simulink model "viikate_rocket"  (R2026b)
settings: Solver=ode4  StopTime=inf  FixedStep=0.001
undefined symbols (not defined in the file or in its folder): Aero, e0_0, e1_0, e2_0, e3_0, gravity, I, N, Newton, Raphson, rho, rp_burn_time_s, rp_canard_area_m2, rp_canard_cl_alpha, rp_cd0, rp_clp, rp_cmq, rp_cn_alpha, rp_cnr, rp_fin_positions_m, rp_frontal_area_m2, rp_gust_seed, rp_gust_variance, rp_ignition_time_s, rp_inertia_empty_kgm2, rp_inertia_full_kgm2, rp_length_m, rp_mass_fuel_kg, rp_mass_full_kg, rp_r_cp_m, rp_roll_ref_length_m, rp_servo_rate_limit_radps, rp_servo_tau_s, rp_thrust_n, rp_thrust_scale, rp_thrust_t_s, rp_wind_model_mps, sharedaeroassertmsg, si, Vsafe, ZYX
libraries: matrix_library x1
(part 1 of 3)
settings Model: Creator=tanel  LastModifiedBy=Minh
settings DataIOCC: ReturnWorkspaceOutputs=off
settings OptimizationCC: DefaultParameterBehavior=Inlined  DifferentSizesBufferReuse=on  EfficientTunableParamExpr=on  EnhancedBackFolding=on  OptimizationCustomize=off  OptimizeBlockOrder=speed  PassReuseOutputArgsAs=Individual arguments  RemoveInternalMemoryZeroInit=on  RemoveRootLevelIOMemoryZeroInit=on
settings DebuggingCC: ParameterTunabilityLossMsg=error
settings HardwareCC: ProdHWDeviceType=Intel->x86-64 (Linux 64)
settings ModelReferenceCC: ModelReferenceMinAlgLoopOccurrences=on
settings SFSimCC: MATLABDynamicMemAlloc=off
settings RTWCC: DataTypeReplacement=CDataTypesFixedWidth  Description=Embedded Coder  GPUComputeCapability=5.0  GenCodeOnly=on  SystemTargetFile=ert.tlc  TemplateMakefile=ert_default_tmf
settings CodeAppCC: ForceParamTrailComments=on  IgnoreCustomStorageClasses=off  InsertBlockDesc=on  OperatorAnnotations=on  SFDataObjDesc=on  SimulinkDataObjDesc=on
settings ERTTargetCC: CombineSignalStateStructs=on  MaxIdInt16=INT16_MAX  MaxIdInt32=INT32_MAX  MaxIdInt64=INT64_MAX  MaxIdInt8=INT8_MAX  MaxIdUint16=UINT16_MAX  MaxIdUint32=UINT32_MAX  MaxIdUint64=UINT64_MAX  MaxIdUint8=UINT8_MAX  MinIdInt16=INT16_MIN  MinIdInt32=INT32_MIN  MinIdInt64=INT64_MIN  MinIdInt8=INT8_MIN  SupportContinuousTime=on

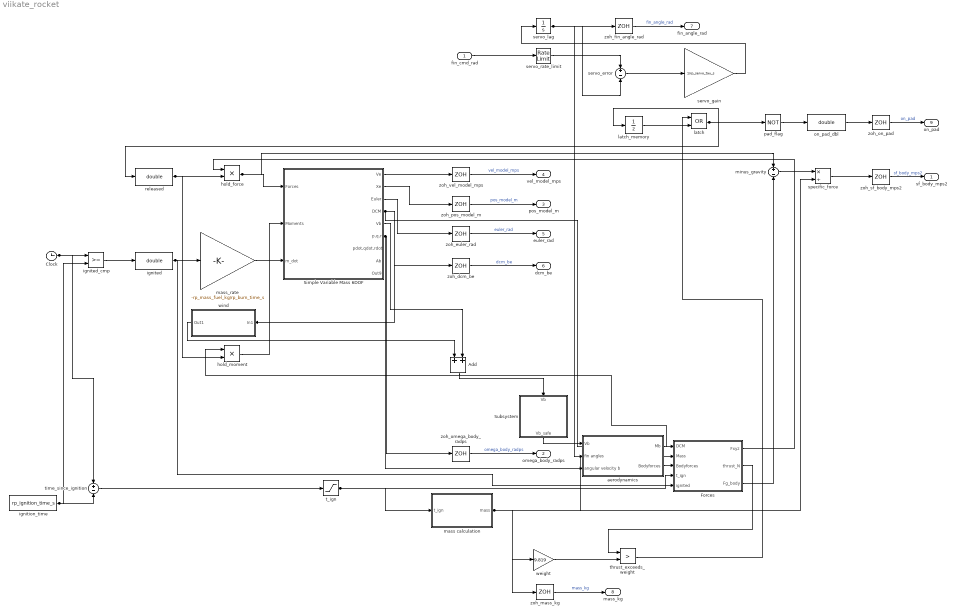
== system viikate_rocket ==
  fin_cmd_rad : Inport  OutDataTypeStr=double  PortDimensions=4  SampleTime=0.001
  Add : Sum
  Clock : Clock
  Forces : Subsystem
  Simple Variable Mass 6DOF : Subsystem  mask(6DOF EoM (Body Axis)){units=Metric (MKS), mtype=Simple Variable, rep=Quaternion, xme_0=[0 50 50], Vm_0=[0 0 0], eul_0=[0 0 0], pm_0=[0 0 0], mass_0=rp_mass_full_kg, mass_e=rp_mass_full_kg - rp_mass_fuel_kg, mass_f=rp_mass_full_kg, inertia=eye(3), inertia_e=rp_inertia_empty_kgm2, inertia_f=rp_inertia_full_kgm2, k_quat=1.0, vre_flag=off, abi_flag=off, aMode=0, xme_statename='', Vm_statename='', eul_statename='', quat_statename='', pm_statename='', mass_statename=''}
      mask prompts: units "shared_aeroblks:sharedaeroblk6dofbody:block6DOFEoMBodyAxisParamUnits"; mtype "shared_aeroblks:sharedaeroblk6dofbody:block6DOFEoMBodyAxisParamMasstype"; rep "shared_aeroblks:sharedaeroblk6dofbody:block6DOFEoMBodyAxisParamRepresentation"; xme_0 "shared_aeroblks:sharedaeroblk6dofbody:block6DOFEoMBodyAxisParamInitialpositionininertialaxesXeYeZe"; Vm_0 "shared_aeroblks:sharedaeroblk6dofbody:block6DOFEoMBodyAxisParamInitialvelocityinbodyaxesUvw"; eul_0 "shared_aeroblks:sharedaeroblk6dofbody:block6DOFEoMBodyAxisParamInitialEulerorientationrollpitchyaw"; pm_0 "shared_aeroblks:sharedaeroblk6dofbody:block6DOFEoMBodyAxisParamInitialbodyrotationratespqr"; mass_0 "shared_aeroblks:sharedaeroblk6dofbody:block6DOFEoMBodyAxisParamInitialmass"; mass_e "shared_aeroblks:sharedaeroblk6dofbody:block6DOFEoMBodyAxisParamEmptymass"; mass_f "shared_aeroblks:sharedaeroblk6dofbody:block6DOFEoMBodyAxisParamFullmass"; inertia "shared_aeroblks:sharedaeroblk6dofbody:block6DOFEoMBodyAxisParamInertia"; inertia_e "shared_aeroblks:sharedaeroblk6dofbody:block6DOFEoMBodyAxisParamEmptyinertiamatrix"; inertia_f "shared_aeroblks:sharedaeroblk6dofbody:block6DOFEoMBodyAxisParamFullinertiamatrix"; k_quat "shared_aeroblks:sharedaeroblk6dofbody:block6DOFEoMBodyAxisParamGainforquaternionnormalization"; vre_flag "shared_aeroblks:sharedaeroblk6dofbody:block6DOFEoMBodyAxisParamIncludemassflowrelativevelocity"; abi_flag "shared_aeroblks:sharedaeroblk6dofbody:inertialAccelFlag"; xme_statename "shared_aeroblks:sharedaeroblk6dofbody:block6DOFEoMStateNamePosition"; Vm_statename "shared_aeroblks:sharedaeroblk6dofbody:block6DOFEoMStateNameVelocity"; eul_statename "shared_aeroblks:sharedaeroblk6dofbody:block6DOFEoMStateNameEulerAngles"; quat_statename "shared_aeroblks:sharedaeroblk6dofbody:block6DOFEoMStateNameQuaternions"; pm_statename "shared_aeroblks:sharedaeroblk6dofbody:block6DOFEoMStateNameRotationRates"; mass_statename "shared_aeroblks:sharedaeroblk6dofbody:block6DOFEoMStateNameMass"
      mask help: shared_aeroblks:sharedaeroblk6dofbody:block6DOFEoMBodyAxisDesc
      mask init:
      | if aerosharedtest(gcb)
      |     ports=aerosharedicon('shared6dofbody','icon');
      | else
      |     ports=sharedautoicon('shared6dofbody','icon');
      | end
      mask Help: eval('aerosharedhelp(''simple_variable_mass_6dof_quaternion'')');
      mask TypeOptions units: shared_aeroblks:sharedaeroblk6dofbody:block6DOFEoMBodyAxisParamComboMetricMKS | shared_aeroblks:sharedaeroblk6dofbody:block6DOFEoMBodyAxisParamComboEnglishVelocityinfts | shared_aeroblks:sharedaeroblk6dofbody:block6DOFEoMBodyAxisParamComboEnglishVelocityinkts
      mask TypeOptions mtype: shared_aeroblks:sharedaeroblk6dofbody:block6DOFEoMBodyAxisParamComboFixed | shared_aeroblks:sharedaeroblk6dofbody:block6DOFEoMBodyAxisParamComboSimpleVariable | shared_aeroblks:sharedaeroblk6dofbody:block6DOFEoMBodyAxisParamComboCustomVariable
      mask Callback mtype:
      | if aerosharedtest(gcb) && builtin('license','test','aerospace_blockset')
      |     aerosharedicon('shared6dofbody');
      | else
      |     sharedautoicon('shared6dofbody');
      | end
      mask TypeOptions rep: shared_aeroblks:sharedaeroblk6dofbody:block6DOFEoMBodyAxisParamComboEulerAngles | shared_aeroblks:sharedaeroblk6dofbody:block6DOFEoMBodyAxisParamComboQuaternion
      mask Callback rep:
      | if aerosharedtest(gcb) && builtin('license','test','aerospace_blockset')
      |     aerosharedicon('shared6dofbody');
      | else
      |     sharedautoicon('shared6dofbody');
      | end
      mask DialogControl Container4 Prompt: shared_aeroblks:sharedaeroblk6dofbody:block6DOFEoMParamTab
      mask DialogControl units Prompt: Units:
      mask DialogControl mtype Prompt: Mass type:
      mask DialogControl rep Prompt: Representation:
      mask DialogControl xme_0 Prompt: Initial position in inertial axes [Xe,Ye,Ze]:
      mask DialogControl Vm_0 Prompt: Initial velocity in body axes [U,v,w]:
      mask DialogControl eul_0 Prompt: Initial Euler orientation [roll, pitch, yaw]:
      mask DialogControl pm_0 Prompt: Initial body rotation rates [p,q,r]:
      mask DialogControl mass_0 Prompt: Initial mass:
      mask DialogControl mass_e Prompt: Empty mass:
      mask DialogControl mass_f Prompt: Full mass:
      mask DialogControl inertia Prompt: Inertia:
      mask DialogControl inertia_e Prompt: Empty inertia matrix:
      mask DialogControl inertia_f Prompt: Full inertia matrix:
      mask DialogControl k_quat Prompt: Gain for quaternion normalization:
      mask DialogControl vre_flag Prompt: Include mass flow relative velocity
      mask DialogControl abi_flag Prompt: Include inertial acceleration
      mask DialogControl Container6 Prompt: shared_aeroblks:sharedaeroblk6dofbody:block6DOFEoMStateAttributesTab
      mask DialogControl Container7 Prompt: shared_aeroblks:sharedaeroblk6dofbody:block6DOFEoMStateNamesGroup
      mask DialogControl xme_statename Prompt: Position: e.g., {'Xe', 'Ye', 'Ze'}
      mask DialogControl Vm_statename Prompt: Velocity: e.g., {'U', 'v', 'w'}
      mask DialogControl eul_statename Prompt: Euler rotation angles: e.g., {'phi', 'theta', 'psi'}
      mask DialogControl quat_statename Prompt: Quaternion vector: e.g., {'qr', 'qi', 'qj', 'qk'}
      mask DialogControl pm_statename Prompt: Body rotation rates: e.g., {'p', 'q', 'r'}
      mask DialogControl mass_statename Prompt: Mass: e.g., 'mass'
      mask Display:
      | port_label(ports(1).type,ports(1).port,ports(1).txt,'texmode','on');
      | port_label(ports(2).type,ports(2).port,ports(2).txt,'texmode','on');
      | port_label(ports(3).type,ports(3).port,ports(3).txt,'texmode','on');
      | port_label(ports(4).type,ports(4).port,ports(4).txt,'texmode','on');
      | port_label(ports(5).type,ports(5).port,ports(5).txt,'texmode','on');
      | port_label(ports(6).type,ports(6).port,ports(6).txt,'texmode','on');
      | port_label(ports(7).type,ports(7).port,ports(7).txt,'texmode','on');
      | port_label(ports(8).type,ports(8).port,ports(8).txt,'texmode','on');
      | port_label(ports(9).type,ports(9).port,ports(9).txt,'texmode','on');
      | port_label(ports(10).type,ports(10).port,ports(10).txt,'texmode','on');
      | port_label(ports(11).type,ports(11).port,ports(11).txt,'texmode','on');
      | port_label(ports(12).type,ports(12).port,ports(12).txt,'texmode','on');
      | port_label(ports(13).type,ports(13).port,ports(13).txt,'texmode','on');
      | port_label(ports(14).type,ports(14).port,ports(14).txt,'texmode','on');
      | port_label(ports(15).type,ports(15).port,ports(15).txt,'texmode','on');
      | port_label(ports(16).type,ports(16).port,ports(16).txt,'texmode','on');
      | port_label(ports(17).type,ports(17).port,ports(17).txt,'texmode','on');
  Subsystem : Subsystem
  aerodynamics : Subsystem
  hold_force : Product
  hold_moment : Product
  ignited : DataTypeConversion  OutDataTypeStr=double  SaturateOnIntegerOverflow=off  RndMeth=Floor
  ignited_cmp : RelationalOperator  OutDataTypeStr=boolean  ZeroCross=off  RndMeth=Simplest  InputSameDT=off
  ignition_time : Constant  Value=rp_ignition_time_s
  latch : Logic  Operator=OR  AllPortsSameDT=off  OutDataTypeStr=boolean
  latch_memory : UnitDelay  InitialCondition=false  SampleTime=0.001
  mass calculation : Subsystem
  mass_rate : Gain  Gain=-rp_mass_fuel_kg/rp_burn_time_s
  minus_gravity : Sum  Inputs=+-
  on_pad_dbl : DataTypeConversion  OutDataTypeStr=double  SaturateOnIntegerOverflow=off  RndMeth=Floor
  pad_flag : Logic  Operator=NOT  AllPortsSameDT=off  OutDataTypeStr=boolean
  released : DataTypeConversion  OutDataTypeStr=double  SaturateOnIntegerOverflow=off  RndMeth=Floor
  servo_error : Sum  Inputs=+-
  servo_gain : Gain  Gain=1/rp_servo_tau_s
  servo_lag : Integrator
  servo_rate_limit : RateLimiter  RisingSlewLimit=rp_servo_rate_limit_radps  FallingSlewLimit=-rp_servo_rate_limit_radps  SampleTimeMode=inherited
  specific_force : Product  Inputs=*/
  t_ign : Saturate  UpperLimit=inf  LowerLimit=0  ZeroCross=off
  thrust_exceeds_weight : RelationalOperator  Operator=>  OutDataTypeStr=boolean  SampleTime=0.001  RndMeth=Simplest  InputSameDT=off
  time_since_ignition : Sum  Inputs=+-
  weight : Gain  Gain=9.819
  wind : Subsystem
  zoh_dcm_be : ZeroOrderHold  SampleTime=0.001
  zoh_euler_rad : ZeroOrderHold  SampleTime=0.001
  zoh_fin_angle_rad : ZeroOrderHold  SampleTime=0.001
  zoh_mass_kg : ZeroOrderHold  SampleTime=0.001
  zoh_omega_body_radps : ZeroOrderHold  SampleTime=0.001
  zoh_on_pad : ZeroOrderHold  SampleTime=0.001
  zoh_pos_model_m : ZeroOrderHold  SampleTime=0.001
  zoh_sf_body_mps2 : ZeroOrderHold  SampleTime=0.001
  zoh_vel_model_mps : ZeroOrderHold  SampleTime=0.001
  sf_body_mps2 : Outport
  omega_body_radps : Outport  Port=2
  pos_model_m : Outport  Port=3
  vel_model_mps : Outport  Port=4
  euler_rad : Outport  Port=5
  dcm_be : Outport  Port=6
  fin_angle_rad : Outport  Port=7
  mass_kg : Outport  Port=8
  on_pad : Outport  Port=9
  wires:
  minus_gravity/1 -> specific_force/1
  pad_flag/1 -> on_pad_dbl/1
  Forces/1(Fxyz) -> hold_force/1
  latch/1 -> pad_flag/1, released/1, latch_memory/1
  thrust_exceeds_weight/1 -> latch/1
  aerodynamics/2(Bodyforces) -> Forces/3(Bodyforces)
  aerodynamics/1(Mb) -> hold_moment/1
  zoh_fin_angle_rad/1 -> fin_angle_rad/1  "fin_angle_rad"
  zoh_mass_kg/1 -> mass_kg/1  "mass_kg"
  Simple Variable Mass 6DOF/1(Ve) -> zoh_vel_model_mps/1
  zoh_on_pad/1 -> on_pad/1  "on_pad"
  Simple Variable Mass 6DOF/2(Xe) -> zoh_pos_model_m/1
  ignition_time/1 -> ignited_cmp/2, time_since_ignition/2
  Simple Variable Mass 6DOF/6(p,q,r) -> zoh_omega_body_radps/1, aerodynamics/3(angular velocity b)
  mass_rate/1 -> Simple Variable Mass 6DOF/3(m_dot)
  hold_force/1 -> Simple Variable Mass 6DOF/1(Forces), minus_gravity/1
  ignited/1 -> mass_rate/1, Forces/5(ignited)
  servo_gain/1 -> servo_lag/1
  time_since_ignition/1 -> t_ign/1
  released/1 -> hold_moment/2, hold_force/2
  Simple Variable Mass 6DOF/3(Euler) -> zoh_euler_rad/1
  Add/1 -> Subsystem/1(Vb)
  on_pad_dbl/1 -> zoh_on_pad/1
  Forces/3(Fg_body) -> minus_gravity/2
  zoh_dcm_be/1 -> dcm_be/1  "dcm_be"
  Clock/1 -> ignited_cmp/1, time_since_ignition/1
  hold_moment/1 -> Simple Variable Mass 6DOF/2(Moments)
  servo_rate_limit/1 -> servo_error/1
  latch_memory/1 -> latch/2
  wind/1(Out1) -> Add/1
  Simple Variable Mass 6DOF/4(DCM) -> zoh_dcm_be/1, Forces/1(DCM), wind/1(In1)
  Simple Variable Mass 6DOF/5(Vb) -> Add/2
  zoh_sf_body_mps2/1 -> sf_body_mps2/1  "sf_body_mps2"
  t_ign/1 -> mass calculation/1(t_ign), Forces/4(t_ign)
  servo_error/1 -> servo_gain/1
  fin_cmd_rad/1 -> servo_rate_limit/1
  specific_force/1 -> zoh_sf_body_mps2/1
  Subsystem/1(Vb_safe) -> aerodynamics/1(Vb)
  zoh_vel_model_mps/1 -> vel_model_mps/1  "vel_model_mps"
  zoh_pos_model_m/1 -> pos_model_m/1  "pos_model_m"
  zoh_euler_rad/1 -> euler_rad/1  "euler_rad"
  zoh_omega_body_radps/1 -> omega_body_radps/1  "omega_body_radps"
  Forces/2(thrust_N) -> thrust_exceeds_weight/1
  mass calculation/1(mass) -> zoh_mass_kg/1, weight/1, Forces/2(Mass), specific_force/2
  servo_lag/1 -> zoh_fin_angle_rad/1, aerodynamics/2(fin angles), servo_error/2
  ignited_cmp/1 -> ignited/1
  weight/1 -> thrust_exceeds_weight/2

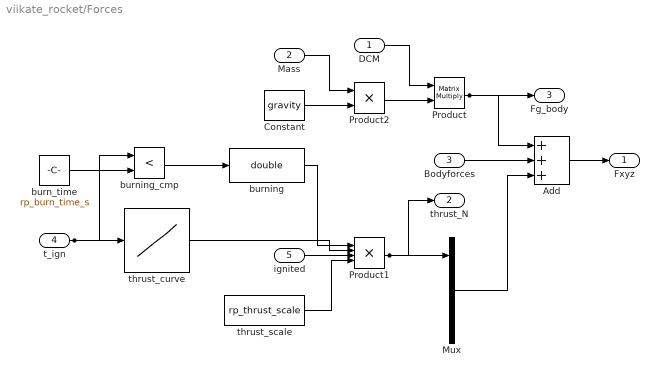
== system viikate_rocket/Forces ==
  DCM : Inport
  Mass : Inport  Port=2
  Bodyforces : Inport  Port=3
  t_ign : Inport  Port=4
  ignited : Inport  Port=5
  Add : Sum  Inputs=+|+|+
  Constant : Constant  Value=gravity  VectorParams1D=off
  Mux : Mux  Inputs=3
  Product : Product  Multiplication=Matrix(*)
  Product1 : Product  Inputs=4
  Product2 : Product
  burn_time : Constant  Value=rp_burn_time_s
  burning : DataTypeConversion  OutDataTypeStr=double  SaturateOnIntegerOverflow=off  RndMeth=Floor
  burning_cmp : RelationalOperator  Operator=<  OutDataTypeStr=boolean  ZeroCross=off  RndMeth=Simplest  InputSameDT=off
  thrust_curve : Lookup_n-D  NumberOfTableDimensions=1  BreakpointsForDimension1=rp_thrust_t_s  Table=rp_thrust_n  ExtrapMethod=Clip  InternalRulePriority=Speed  RndMeth=Simplest
  thrust_scale : Constant  Value=rp_thrust_scale
  Fxyz : Outport
  thrust_N : Outport  Port=2
  Fg_body : Outport  Port=3
  wires:
  Add/1 -> Fxyz/1
  Mux/1 -> Add/3
  burn_time/1 -> burning_cmp/2
  burning/1 -> Product1/1
  Bodyforces/1 -> Add/2
  t_ign/1 -> burning_cmp/1, thrust_curve/1
  Product1/1 -> thrust_N/1, Mux/1
  Product/1 -> Fg_body/1, Add/1
  burning_cmp/1 -> burning/1
  Mass/1 -> Product2/1
  Product2/1 -> Product/2
  Constant/1 -> Product2/2
  thrust_curve/1 -> Product1/2
  ignited/1 -> Product1/3
  thrust_scale/1 -> Product1/4
  DCM/1 -> Product/1

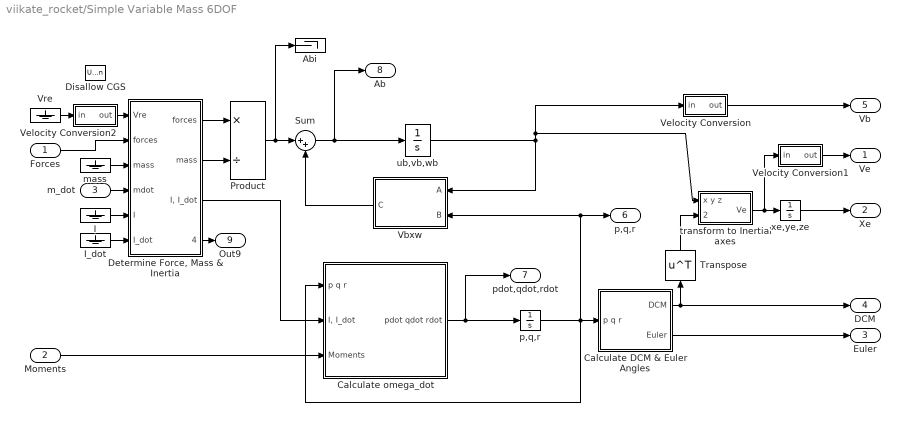
== system viikate_rocket/Simple Variable Mass 6DOF ==
  Forces : Inport  OutDataTypeStr=double  Unit=N  PortDimensions=3
  Moments : Inport  Port=2  OutDataTypeStr=double  Unit=N*m  PortDimensions=3
  m_dot : Inport  Port=3  Unit=kg/s
  Abi : Terminator
  Calculate DCM & Euler Angles : Subsystem  mask(DCM & Euler Angles (Quaternion)){aMode=aMode}
      mask init:
      | if aerosharedtest(gcb)
      |     aerosharedicon('shared');
      | else
      |     sharedautoicon('shared');
      | end
  Calculate omega_dot : Subsystem  mask{aMode=aMode}
      mask init:
      | if aerosharedtest(gcb)
      |     aerosharedicon('shared');
      | else
      |     sharedautoicon('shared');
      | end
  "Determine Force, Mass & Inertia" : Subsystem  mask(Mass & Inertia (simple)){aMode=aMode}
      mask init:
      | if aerosharedtest(gcb)
      |     aerosharedicon('shared');
      | else
      |     sharedautoicon('shared');
      | end
  Disallow CGS : UnitConfiguration  UnitSystemsStr=English,SI,SI (extended)  AllowAllUnitSystems=off
  I : Ground
  I_dot : Ground
  Product : Product  Inputs=*/  SaturateOnIntegerOverflow=on  OutDataTypeStr=Inherit: Same as first input
  Sum : Sum  Inputs=|++  SaturateOnIntegerOverflow=on
  Transpose : Math  Operator=transpose  SignedPower=on
  Vbxw : Subsystem  mask(CrossProduct){aMode=aMode}
      mask help: shared_aeroblks:sharedaeroblkutil:blockCrossProductDesc
      mask init:
      | if aerosharedtest(gcb)
      |     aerosharedicon('shared');
      | else
      |     sharedautoicon('shared');
      | end
      mask Help: eval('if license(''test'',''Aerospace_Blockset'')aerosharedhelp(''threebythree_cross_product'');elseif license(''test'',''Powertrain_Blockset'')sharedautohelp(''threebythree_cross_product'');end')
      mask Display:
      | text(.5,.5,'Cross\nProduct\nC = AxB', ...
      | 	'HorizontalAlignment','Center',...
      | 	'VerticalAlignment','middle')
  Velocity Conversion : Subsystem
  Velocity Conversion1 : Subsystem
  Velocity Conversion2 : Subsystem
  Vre : Ground
  mass : Ground
  "p,q,r " : Integrator  InitialCondition=pm_0  ContinuousStateAttributes=pm_statename
  "transform to Inertial axes " : Subsystem  mask(Vector Transformation){}
      mask Display: disp('L_EB')
  ub,vb,wb : Integrator  InitialCondition=Vm_0  ContinuousStateAttributes=Vm_statename
  xe,ye,ze : Integrator  InitialCondition=xme_0  ContinuousStateAttributes=xme_statename
  Ve : Outport  OutDataTypeStr=double  Unit=m/s  VectorParamsAs1DForOutWhenUnconnected=off
  Xe : Outport  Port=2  OutDataTypeStr=double  Unit=m  VectorParamsAs1DForOutWhenUnconnected=off
  Euler : Outport  Port=3  OutDataTypeStr=double  Unit=rad  VectorParamsAs1DForOutWhenUnconnected=off
  DCM : Outport  Port=4  OutDataTypeStr=double  Unit=1  VectorParamsAs1DForOutWhenUnconnected=off
  Vb : Outport  Port=5  OutDataTypeStr=double  Unit=m/s  VectorParamsAs1DForOutWhenUnconnected=off
  p,q,r : Outport  Port=6  OutDataTypeStr=double  Unit=rad/s  VectorParamsAs1DForOutWhenUnconnected=off
  pdot,qdot,rdot : Outport  Port=7  OutDataTypeStr=double  Unit=rad/s^2  VectorParamsAs1DForOutWhenUnconnected=off
  Ab : Outport  Port=8  OutDataTypeStr=double  Unit=m/s^2  VectorParamsAs1DForOutWhenUnconnected=off
  Out9 : Outport  Port=9  Unit=1
  wires:
  Velocity Conversion1/1(out) -> Ve/1
  Sum/1 -> Ab/1, ub,vb,wb/1
  ub,vb,wb/1 -> Vbxw/1(A), Velocity Conversion/1(in), "transform to Inertial axes "/1(x y z)
  Velocity Conversion/1(out) -> Vb/1
  Velocity Conversion2/1(out) -> "Determine Force, Mass & Inertia"/1(Vre)
  Vre/1 -> Velocity Conversion2/1(in)
  "Determine Force, Mass & Inertia"/1("forces ") -> Product/1
  I_dot/1 -> "Determine Force, Mass & Inertia"/6(I_dot)
  I/1 -> "Determine Force, Mass & Inertia"/5(I)
  Calculate omega_dot/1(pdot qdot rdot) -> "p,q,r "/1, pdot,qdot,rdot/1
  "Determine Force, Mass & Inertia"/4(tank limit) -> Out9/1
  m_dot/1 -> "Determine Force, Mass & Inertia"/4(mdot)
  "Determine Force, Mass & Inertia"/2(mass) -> Product/2
  mass/1 -> "Determine Force, Mass & Inertia"/3("mass ")
  Transpose/1 -> "transform to Inertial axes "/2(transform coefficients)
  Calculate DCM & Euler Angles/1(DCM) -> Transpose/1, DCM/1
  Product/1 -> Sum/1, Abi/1
  Forces/1 -> "Determine Force, Mass & Inertia"/2(forces)
  Moments/1 -> Calculate omega_dot/3(Moments)
  "p,q,r "/1 -> Calculate DCM & Euler Angles/1(p q r), Calculate omega_dot/1(p q r), p,q,r/1, Vbxw/2(B)
  "transform to Inertial axes "/1(Ve) -> xe,ye,ze/1, Velocity Conversion1/1(in)
  xe,ye,ze/1 -> Xe/1
  Vbxw/1(C) -> Sum/2
  Calculate DCM & Euler Angles/2(Euler) -> Euler/1
  "Determine Force, Mass & Inertia"/3("I, I_dot") -> Calculate omega_dot/2("I, I_dot")

== system viikate_rocket/Subsystem ==
  Vb : Inport
  Abs : Abs  SaturateOnIntegerOverflow=off
  Constant3 : Constant  Value=Vsafe
  Demux : Demux  Outputs=3
  Mux : Mux  Inputs=3
  Switch2 : Switch  Threshold=Vsafe  SaturateOnIntegerOverflow=off  InputSameDT=off
  Vb_safe : Outport
  wires:
  Vb/1 -> Demux/1
  Abs/1 -> Switch2/2
  Demux/2 -> Mux/2
  Demux/3 -> Mux/3
  Switch2/1 -> Mux/1
  Mux/1 -> Vb_safe/1
  Demux/1 -> Switch2/1, Abs/1
  Constant3/1 -> Switch2/3

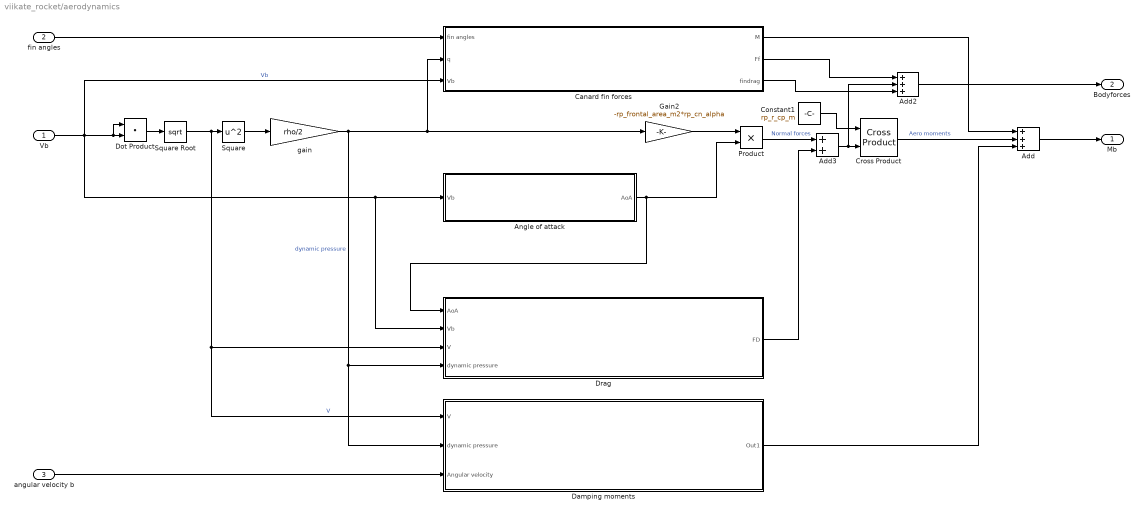
== system viikate_rocket/aerodynamics ==
  Vb : Inport
  fin angles : Inport  Port=2
  angular velocity b : Inport  Port=3
  Add : Sum  Inputs=+++
  Add2 : Sum  Inputs=+++
  Add3 : Sum
  Angle of attack : Subsystem
  Canard fin forces : Subsystem
  Constant1 : Constant  Value=rp_r_cp_m
  Cross Product : matrix_library/Cross Product
  Damping moments : Subsystem
  Dot Product : DotProduct  OutDataTypeStr=Inherit: Inherit via internal rule
  Drag : Subsystem
  Gain2 : Gain  Gain=-rp_frontal_area_m2*rp_cn_alpha
  Product : Product
  Square : Math  Operator=square
  Square Root : Sqrt
  gain : Gain  Gain=rho/2
  Mb : Outport
  Bodyforces : Outport  Port=2
  wires:
  Gain2/1 -> Product/1
  Constant1/1 -> Cross Product/1
  Product/1 -> Add3/1  "Normal forces"
  Cross Product/1 -> Add/2  "Aero moments"
  Add/1 -> Mb/1
  Add2/1 -> Bodyforces/1
  Canard fin forces/2(Ff) -> Add2/1
  Add3/1 -> Add2/2, Cross Product/2
  Vb/1 -> Canard fin forces/3(Vb), Dot Product/1, Dot Product/2, Angle of attack/1(Vb), Drag/2(Vb)  "Vb"
  Square/1 -> gain/1
  Square Root/1 -> Damping moments/1(V), Drag/3(V), Square/1  "V"
  Dot Product/1 -> Square Root/1
  gain/1 -> Damping moments/2(dynamic pressure), Drag/4(dynamic pressure), Canard fin forces/2(q), Gain2/1  "dynamic pressure"
  fin angles/1 -> Canard fin forces/1(fin angles)
  Canard fin forces/1(M) -> Add/1
  Drag/1(FD) -> Add3/2
  Angle of attack/1(AoA) -> Product/2, Drag/1(AoA)
  angular velocity b/1 -> Damping moments/3(Angular velocity)
  Damping moments/1(Out1) -> Add/3
  Canard fin forces/3(findrag) -> Add2/3

== system viikate_rocket/mass calculation ==
  t_ign : Inport
  Add : Sum
  Constant1 : Constant  Value=rp_mass_full_kg
  Constant2 : Constant  Value=-rp_mass_fuel_kg/rp_burn_time_s
  Product : Product
  Saturation : Saturate  UpperLimit=rp_mass_full_kg  LowerLimit=rp_mass_full_kg - rp_mass_fuel_kg
  mass : Outport
  wires:
  Add/1 -> Saturation/1
  Product/1 -> Add/2
  Saturation/1 -> mass/1
  t_ign/1 -> Product/2
  Constant1/1 -> Add/1
  Constant2/1 -> Product/1

== system viikate_rocket/wind ==
  In1 : Inport
  Constant3 : Constant  Value=0
  Gain : Gain  Gain=-1
  Integrator : Integrator  InitialCondition=rp_wind_model_mps
  Matrix Multiply : Product  Multiplication=Matrix(*)
  Mux : Mux  Inputs=3
  Random Number1 : RandomNumber  Variance=rp_gust_variance  Seed=rp_gust_seed(1)  SampleTime=0.01
  Random Number2 : RandomNumber  Variance=rp_gust_variance  Seed=rp_gust_seed(2)  SampleTime=0.01
  Out1 : Outport
  wires:
  Mux/1 -> Integrator/1
  Constant3/1 -> Mux/1
  Gain/1 -> Matrix Multiply/2
  Random Number1/1 -> Mux/2
  Random Number2/1 -> Mux/3
  Integrator/1 -> Gain/1
  Matrix Multiply/1 -> Out1/1
  In1/1 -> Matrix Multiply/1

== system viikate_rocket/Simple Variable Mass 6DOF/Calculate DCM & Euler Angles ==
  p q r : Inport  OutDataTypeStr=double
  Initial Euler Angles : Constant  Value=eul_0
  Quaternions to Direction Cosine Matrix : Subsystem  mask(Quaternion2DCM){aMode=aMode}
      mask help: shared_aeroblks:sharedaeroblktransform:blockQuaternion2DCMDesc
      mask init:
      | if aerosharedtest(gcb)
      |     ports=aerosharedicon('shared');
      | else
      |     ports=sharedautoicon('shared');
      | end
      mask Help: eval('if license(''test'',''Aerospace_Blockset'')aerosharedhelp(''quaternions_to_direction_cosine_matrix'');elseif license(''test'',''Powertrain_Blockset'')sharedautohelp(''quaternions_to_direction_cosine_matrix'');end')
      mask Display:
      | port_label('input',1,'q','texmode','on')
      | port_label('output',1,'DCM_{be}','texmode','on')
  Quaternions to Rotation Angles : Subsystem  mask(Quat2Ang){rotationOrder=ZYX, aMode=aMode}
      mask prompts: rotationOrder "shared_aeroblks:sharedaeroblktransform:blockDCM2AngParamRotationOrder"
      mask help: shared_aeroblks:sharedaeroblktransform:blockQuat2AngDesc
      settings: AttributesFormatString=Rotation Order: %<rotationOrder>
      mask Help: eval('if license(''test'',''Aerospace_Blockset'')aerosharedhelp(''quaternions_to_rotation_angles'');elseif license(''test'',''Powertrain_Blockset'')sharedautohelp(''quaternions_to_rotation_angles'');end')
      mask TypeOptions rotationOrder: DCM2Ang/rotationOrder
      mask DialogControl rotationOrder Prompt: Rotation order:
      mask Display:
      | port_label('input',1,'q','texmode','on')
      | port_label('output',1,'[R_1,R_2,R_3]','texmode','on')
  Rotation Angles to Quaternions : Subsystem  mask(Ang2Quat){rotationOrder=ZYX, aMode=aMode}
      mask prompts: rotationOrder "shared_aeroblks:sharedaeroblktransform:blockAng2QuatParamRotationOrder"
      mask help: shared_aeroblks:sharedaeroblktransform:blockAng2QuatDesc
      mask init:
      | if aerosharedtest(gcb)
      |     ports=aerosharedicon('sharedang2quat');
      | else
      |     ports=sharedautoicon('sharedang2quat');
      | end
      settings: AttributesFormatString=Rotation Order: %<rotationOrder>
      mask Help: eval('if license(''test'',''Aerospace_Blockset'')aerosharedhelp(''rotation_angles_to_quaternions'');elseif license(''test'',''Powertrain_Blockset'')sharedautohelp(''rotation_angles_to_quaternions'');end')
      mask TypeOptions rotationOrder: shared_aeroblks:sharedaeroblktransform:blockParamComboZYX | shared_aeroblks:sharedaeroblktransform:blockParamComboZYZ | shared_aeroblks:sharedaeroblktransform:blockParamComboZXY | shared_aeroblks:sharedaeroblktransform:blockParamComboZXZ | shared_aeroblks:sharedaeroblktransform:blockParamComboYXZ | shared_aeroblks:sharedaeroblktransform:blockParamComboYXY | shared_aeroblks:sharedaeroblktransform:blockParamComboYZX | shared_aeroblks:sharedaeroblktransform:blockParamComboYZY | shared_aeroblks:sharedaeroblktransform:blockParamComboXYZ | shared_aeroblks:sharedaeroblktransform:blockParamComboXYX | shared_aeroblks:sharedaeroblktransform:blockParamComboXZY | shared_aeroblks:sharedaeroblktransform:blockParamComboXZX
      mask DialogControl rotationOrder Prompt: Rotation order:
      mask Display:
      | port_label('input',1,'[R_1,R_2,R_3]','texmode','on')
      | port_label('output',1,'q','texmode','on')
  Selector : Selector  InputPortWidth=3  IndexOptions=Index vector (dialog)  Indices=[3 2 1]  OutputSizes=1  RuntimeRangeChecks=off
  Selector1 : Selector  InputPortWidth=3  IndexOptions=Index vector (dialog)  Indices=[3 2 1]  OutputSizes=1  RuntimeRangeChecks=off
  q0 q1 q2 q3 : Integrator  InitialConditionSource=external  InitialCondition=[e0_0 e1_0 e2_0 e3_0]  ContinuousStateAttributes=quat_statename
  qdot : Subsystem
  DCM : Outport  OutDataTypeStr=double  VectorParamsAs1DForOutWhenUnconnected=off
  Euler : Outport  Port=2  OutDataTypeStr=double  VectorParamsAs1DForOutWhenUnconnected=off
  wires:
  Selector1/1 -> Rotation Angles to Quaternions/1("R1, R2, R3")
  Selector/1 -> Euler/1
  Quaternions to Rotation Angles/1(R1,R2,R3) -> Selector/1
  Quaternions to Direction Cosine Matrix/1(DCM) -> DCM/1
  p q r/1 -> qdot/1(p q r)
  Initial Euler Angles/1 -> Selector1/1
  Rotation Angles to Quaternions/1(Quat) -> q0 q1 q2 q3/2
  q0 q1 q2 q3/1 -> qdot/2(q0 q1 q2 q3), Quaternions to Rotation Angles/1(q), Quaternions to Direction Cosine Matrix/1(Quat)
  qdot/1(qdot) -> q0 q1 q2 q3/1

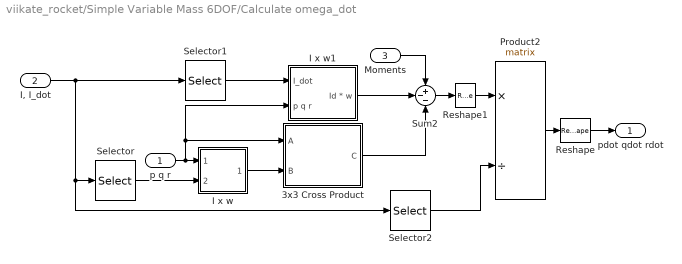
== system viikate_rocket/Simple Variable Mass 6DOF/Calculate omega_dot ==
  p q r : Inport  OutDataTypeStr=double
  "I, I_dot" : Inport  Port=2  OutDataTypeStr=double
  Moments : Inport  Port=3  OutDataTypeStr=double
  3x3 Cross Product : Subsystem  mask(CrossProduct){aMode=aMode}
      mask help: shared_aeroblks:sharedaeroblkutil:blockCrossProductDesc
      mask init:
      | if aerosharedtest(gcb)
      |     aerosharedicon('shared');
      | else
      |     sharedautoicon('shared');
      | end
      mask Help: eval('if license(''test'',''Aerospace_Blockset'')aerosharedhelp(''threebythree_cross_product'');elseif license(''test'',''Powertrain_Blockset'')sharedautohelp(''threebythree_cross_product'');end')
      mask Display:
      | text(.5,.5,'Cross\nProduct\nC = AxB', ...
      | 	'HorizontalAlignment','Center',...
      | 	'VerticalAlignment','middle')
  I x w : Subsystem
  I x w1 : Subsystem
  Product2 : Product  Inputs=*/  Multiplication=Matrix(*)  SaturateOnIntegerOverflow=on  OutDataTypeStr=Inherit: Same as first input
  Reshape : Reshape
  Reshape1 : Reshape  OutputDimensionality=Row vector (2-D)
  Selector : Selector  NumberOfDimensions=2  InputPortWidth=2  IndexOptions=Index vector (dialog),Select all  Indices=1:3,-1  OutputSizes=1  RuntimeRangeChecks=off
  Selector1 : Selector  NumberOfDimensions=2  InputPortWidth=2  IndexOptions=Index vector (dialog),Select all  Indices=4:6,-1  OutputSizes=1  RuntimeRangeChecks=off
  Selector2 : Selector  NumberOfDimensions=2  InputPortWidth=2  IndexOptions=Index vector (dialog),Select all  Indices=1:3,-1  OutputSizes=1  RuntimeRangeChecks=off
  Sum2 : Sum  Inputs=+--  SaturateOnIntegerOverflow=on
  pdot qdot rdot : Outport  OutDataTypeStr=double  VectorParamsAs1DForOutWhenUnconnected=off
  wires:
  Reshape1/1 -> Product2/1
  I x w/1(I * w) -> 3x3 Cross Product/2(B)
  3x3 Cross Product/1(C) -> Sum2/3
  Selector1/1 -> I x w1/1(I_dot)
  I x w1/1(Id * w) -> Sum2/2
  Moments/1 -> Sum2/1
  Sum2/1 -> Reshape1/1
  Product2/1 -> Reshape/1
  p q r/1 -> I x w1/2(p q r), 3x3 Cross Product/1(A), I x w/1(p q r)
  "I, I_dot"/1 -> Selector1/1, Selector2/1, Selector/1
  Selector2/1 -> Product2/2
  Selector/1 -> I x w/2(Inertia)
  Reshape/1 -> pdot qdot rdot/1

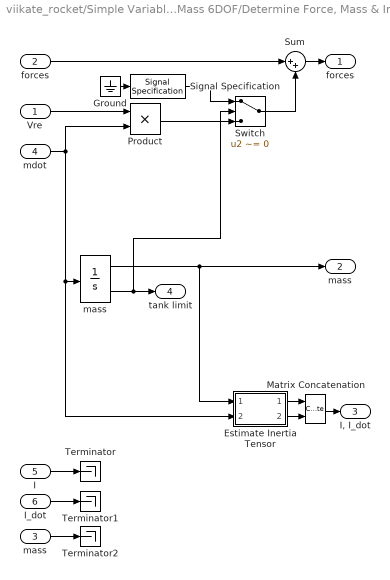
== system viikate_rocket/Simple Variable Mass 6DOF/Determine Force, Mass & Inertia ==
  Vre : Inport  OutDataTypeStr=double
  forces : Inport  Port=2  OutDataTypeStr=double
  "mass " : Inport  Port=3  OutDataTypeStr=double
  mdot : Inport  Port=4  OutDataTypeStr=double
  I : Inport  Port=5  OutDataTypeStr=double
  I_dot : Inport  Port=6  OutDataTypeStr=double
  Estimate Inertia Tensor : Subsystem  mask(Estimate Inertia Tensor){fmass=mass_f, emass=mass_e, fI=inertia_f, eI=inertia_e, aMode=aMode}
      mask prompts: fmass "shared_aeroblks:sharedaeroblkbdyn:blockEstimateInertiaTensorParamFullmass"; emass "shared_aeroblks:sharedaeroblkbdyn:blockEstimateInertiaTensorParamEmptymass"; fI "shared_aeroblks:sharedaeroblkbdyn:blockEstimateInertiaTensorParamFullinertiamatrix"; eI "shared_aeroblks:sharedaeroblkbdyn:blockEstimateInertiaTensorParamEmptyinertiamatrix"
      mask help: shared_aeroblks:sharedaeroblkbdyn:blockEstimateInertiaTensorDesc
      mask init:
      | if aerosharedtest(gcb)
      |     aerosharedicon('shared');
      | else
      |     sharedautoicon('shared');
      | end
      | I(:,:,1)=eI;
      | I(:,:,2)=fI;
      mask Help: eval('if license(''test'',''Aerospace_Blockset'')aerosharedhelp;elseif license(''test'',''Powertrain_Blockset'')sharedautohelp;end')
      mask DialogControl fmass Prompt: Full mass:
      mask DialogControl emass Prompt: Empty mass:
      mask DialogControl fI Prompt: Full inertia matrix:
      mask DialogControl eI Prompt: Empty inertia matrix:
      mask Display:
      | port_label('input',1,'mass','texmode','on');
      | port_label('input',2,'dm/dt','texmode','on');
      | port_label('output',1,'I','texmode','on');
      | port_label('output',2,'dI/dt','texmode','on');
      | if aerosharedtest(gcb) && license('test','Aerospace_Blockset')
      |     p=aerosharedimage('inertia',gcbh);
      | elseif license('test','Powertrain_Blockset')
      |     p=sharedautoimage('inertia',gcbh);
      | end
      | patch(p.xp,p.yp);
      | patch(p.xp2,p.yp2);
  Ground : Ground
  Matrix Concatenation : Concatenate  Mode=Multidimensional array
  Product : Product
  Signal Specification : SignalSpecification  OutDataTypeStr=double
  Sum : Sum  Inputs=|++  SaturateOnIntegerOverflow=on
  Switch : Switch  Criteria=u2 ~= 0  SaturateOnIntegerOverflow=off  InputSameDT=off
  Terminator : Terminator
  Terminator1 : Terminator
  Terminator2 : Terminator
  "mass  " : Integrator  InitialCondition=mass_0  LimitOutput=on  UpperSaturationLimit=mass_f  LowerSaturationLimit=mass_e  ShowSaturationPort=on  ContinuousStateAttributes=mass_statename
  "forces " : Outport  OutDataTypeStr=double  PortDimensions=3  VectorParamsAs1DForOutWhenUnconnected=off
  mass : Outport  Port=2  OutDataTypeStr=double  VectorParamsAs1DForOutWhenUnconnected=off
  "I, I_dot" : Outport  Port=3  OutDataTypeStr=double  VectorParamsAs1DForOutWhenUnconnected=off
  tank limit : Outport  Port=4  OutDataTypeStr=double  VectorParamsAs1DForOutWhenUnconnected=off
  wires:
  Signal Specification/1 -> Switch/1
  Ground/1 -> Signal Specification/1
  Product/1 -> Switch/3
  Vre/1 -> Product/1
  Switch/1 -> Sum/2
  Sum/1 -> "forces "/1
  forces/1 -> Sum/1
  "mass "/1 -> Terminator2/1
  I_dot/1 -> Terminator1/1
  Matrix Concatenation/1 -> "I, I_dot"/1
  Estimate Inertia Tensor/2(I_dot) -> Matrix Concatenation/2
  I/1 -> Terminator/1
  Estimate Inertia Tensor/1(Inertia) -> Matrix Concatenation/1
  mdot/1 -> "mass  "/1, Estimate Inertia Tensor/2(M_dot), Product/2
  "mass  "/1 -> mass/1, Estimate Inertia Tensor/1(Mass)
  "mass  "/2 -> tank limit/1, Switch/2

== system viikate_rocket/Simple Variable Mass 6DOF/Vbxw ==
  A : Inport
  B : Inport  Port=2
  "A " : InportShadow
  "B " : InportShadow  Port=2
  Subsystem : Subsystem
  Subsystem1 : Subsystem
  Sum : Sum  Inputs=+|-  InputSameDT=on  SaturateOnIntegerOverflow=on  OutDataTypeStr=Inherit: Same as first input
  C : Outport  VectorParamsAs1DForOutWhenUnconnected=off
  wires:
  "B "/1 -> Subsystem1/2(B)
  "A "/1 -> Subsystem1/1(A)
  Sum/1 -> C/1
  B/1 -> Subsystem/2(B)
  A/1 -> Subsystem/1(A)
  Subsystem/1(Out1) -> Sum/1
  Subsystem1/1(Out1) -> Sum/2

== system viikate_rocket/Simple Variable Mass 6DOF/Velocity Conversion ==
  in : Inport  Unit=m/s
  Unit Conversion : UnitConversion
  out : Outport  VectorParamsAs1DForOutWhenUnconnected=off
  wires:
  Unit Conversion/1 -> out/1
  in/1 -> Unit Conversion/1

== system viikate_rocket/Simple Variable Mass 6DOF/Velocity Conversion1 ==
  in : Inport  Unit=m/s
  Unit Conversion : UnitConversion
  out : Outport  VectorParamsAs1DForOutWhenUnconnected=off
  wires:
  Unit Conversion/1 -> out/1
  in/1 -> Unit Conversion/1

== system viikate_rocket/Simple Variable Mass 6DOF/Velocity Conversion2 ==
  in : Inport  OutDataTypeStr=double  Unit=m/s
  Unit Conversion : UnitConversion
  out : Outport  Unit=m/s  VectorParamsAs1DForOutWhenUnconnected=off
  wires:
  Unit Conversion/1 -> out/1
  in/1 -> Unit Conversion/1

== system viikate_rocket/Simple Variable Mass 6DOF/transform to Inertial axes  ==
  x y z : Inport
  transform coefficients : Inport  Port=2
  Product : Product  Multiplication=Matrix(*)  InputSameDT=on  SaturateOnIntegerOverflow=on  OutDataTypeStr=Inherit: Same as first input
  Reshape1 : Reshape  OutputDimensionality=Column vector (2-D)
  Reshape2 : Reshape
  Ve : Outport  VectorParamsAs1DForOutWhenUnconnected=off
  wires:
  Reshape2/1 -> Ve/1
  Reshape1/1 -> Product/2
  x y z/1 -> Reshape1/1
  transform coefficients/1 -> Product/1
  Product/1 -> Reshape2/1

== system viikate_rocket/aerodynamics/Angle of attack ==
  Vb : Inport
  Atan : Trigonometry  Operator=atan
  Constant2 : Constant  Value=0
  Demux : Demux  Outputs=3
  Divide : Product  Inputs=/*  OutMin=[-pi]  OutMax=[pi]
  Mux : Mux  Inputs=3
  AoA : Outport
  wires:
  Mux/1 -> Divide/2
  Demux/2 -> Mux/2
  Demux/3 -> Mux/3
  Divide/1 -> Atan/1  "AoA (small a)"
  Constant2/1 -> Mux/1
  Atan/1 -> AoA/1  "AoA"
  Demux/1 -> Divide/1
  Vb/1 -> Demux/1

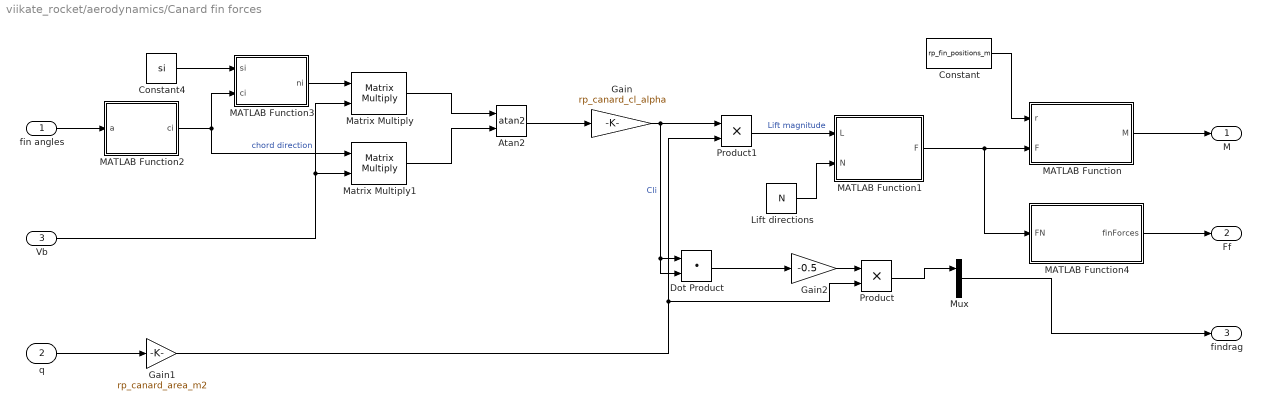
== system viikate_rocket/aerodynamics/Canard fin forces ==
  fin angles : Inport
  q : Inport  Port=2
  Vb : Inport  Port=3
  Atan2 : Trigonometry  Operator=atan2
  Constant : Constant  Value=rp_fin_positions_m
  Constant4 : Constant  Value=si
  Dot Product : DotProduct  OutDataTypeStr=Inherit: Inherit via internal rule
  Gain : Gain  Gain=rp_canard_cl_alpha
  Gain1 : Gain  Gain=rp_canard_area_m2
  Gain2 : Gain  Gain=-0.5
  Lift directions : Constant  Value=N
  MATLAB Function : MATLAB Function  TreatAsAtomicUnit=on
  MATLAB Function1 : MATLAB Function  TreatAsAtomicUnit=on
  MATLAB Function2 : MATLAB Function  TreatAsAtomicUnit=on
  MATLAB Function3 : MATLAB Function  TreatAsAtomicUnit=on
  MATLAB Function4 : MATLAB Function  TreatAsAtomicUnit=on
  Matrix Multiply : Product  Multiplication=Matrix(*)
  Matrix Multiply1 : Product  Multiplication=Matrix(*)
  Mux : Mux  Inputs=3
  Product : Product
  Product1 : Product
  M : Outport
  Ff : Outport  Port=2
  findrag : Outport  Port=3
  wires:
  Constant4/1 -> MATLAB Function3/1(si)
  MATLAB Function1/1(F) -> MATLAB Function4/1(FN), MATLAB Function/2(F)
  Matrix Multiply/1 -> Atan2/1
  Atan2/1 -> Gain/1
  Constant/1 -> MATLAB Function/1(r)
  Lift directions/1 -> MATLAB Function1/2(N)
  Product1/1 -> MATLAB Function1/1(L)  "Lift magnitude"
  Gain/1 -> Product1/1, Dot Product/2, Dot Product/1  "Cli"
  MATLAB Function2/1(ci) -> MATLAB Function3/2(ci), Matrix Multiply1/1  "chord direction"
  Vb/1 -> Matrix Multiply/2, Matrix Multiply1/2
  Matrix Multiply1/1 -> Atan2/2
  fin angles/1 -> MATLAB Function2/1(a)
  MATLAB Function3/1(ni) -> Matrix Multiply/1
  MATLAB Function/1(M) -> M/1
  q/1 -> Gain1/1
  Gain1/1 -> Product/2, Product1/2
  MATLAB Function4/1(finForces) -> Ff/1
  Gain2/1 -> Product/1
  Product/1 -> Mux/1
  Mux/1 -> findrag/1
  Dot Product/1 -> Gain2/1

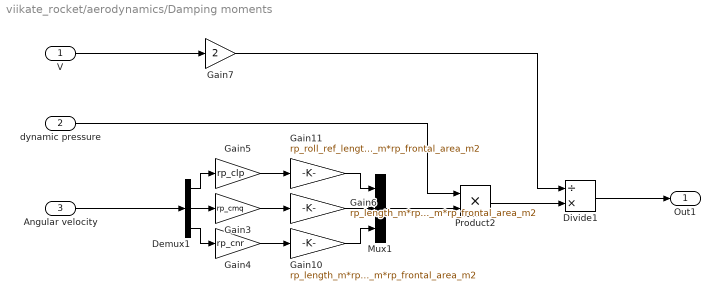
== system viikate_rocket/aerodynamics/Damping moments ==
  V : Inport
  dynamic pressure : Inport  Port=2
  Angular velocity : Inport  Port=3
  Demux1 : Demux  Outputs=3
  Divide1 : Product  Inputs=/*  SaturateOnIntegerOverflow=on
  Gain10 : Gain  Gain=rp_length_m*rp_length_m*rp_frontal_area_m2
  Gain11 : Gain  Gain=rp_roll_ref_length_m*rp_roll_ref_length_m*rp_frontal_area_m2
  Gain3 : Gain  Gain=rp_cmq
  Gain4 : Gain  Gain=rp_cnr
  Gain5 : Gain  Gain=rp_clp
  Gain6 : Gain  Gain=rp_length_m*rp_length_m*rp_frontal_area_m2
  Gain7 : Gain  Gain=2
  Mux1 : Mux  Inputs=3
  Product2 : Product
  Out1 : Outport
  wires:
  Mux1/1 -> Product2/2
  Gain11/1 -> Mux1/1
  Demux1/1 -> Gain5/1
  Demux1/2 -> Gain3/1
  Gain7/1 -> Divide1/1
  Product2/1 -> Divide1/2
  Demux1/3 -> Gain4/1
  Gain3/1 -> Gain6/1
  Gain5/1 -> Gain11/1
  Gain4/1 -> Gain10/1
  Gain10/1 -> Mux1/3
  Angular velocity/1 -> Demux1/1
  Gain6/1 -> Mux1/2
  Divide1/1 -> Out1/1
  V/1 -> Gain7/1
  dynamic pressure/1 -> Product2/1

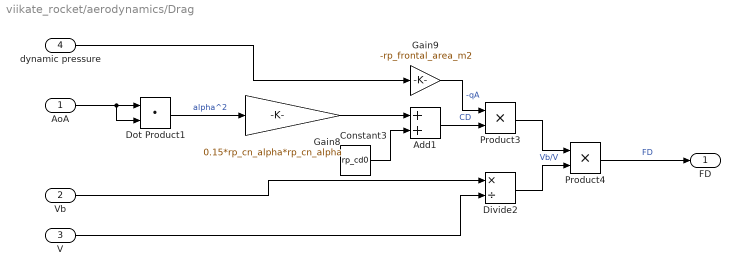
== system viikate_rocket/aerodynamics/Drag ==
  AoA : Inport
  Vb : Inport  Port=2
  V : Inport  Port=3
  dynamic pressure : Inport  Port=4
  Add1 : Sum
  Constant3 : Constant  Value=rp_cd0
  Divide2 : Product  Inputs=*/  SaturateOnIntegerOverflow=on
  Dot Product1 : DotProduct  OutDataTypeStr=Inherit: Inherit via internal rule
  Gain8 : Gain  Gain=0.15*rp_cn_alpha*rp_cn_alpha
  Gain9 : Gain  Gain=-rp_frontal_area_m2
  Product3 : Product
  Product4 : Product
  FD : Outport
  wires:
  AoA/1 -> Dot Product1/2, Dot Product1/1
  Product3/1 -> Product4/1
  Product4/1 -> FD/1  "FD"
  Vb/1 -> Divide2/1
  Divide2/1 -> Product4/2  "Vb/V"
  Constant3/1 -> Add1/2
  Add1/1 -> Product3/2  "CD"
  Gain9/1 -> Product3/1  "-qA"
  Gain8/1 -> Add1/1
  Dot Product1/1 -> Gain8/1  "alpha^2"
  dynamic pressure/1 -> Gain9/1
  V/1 -> Divide2/2

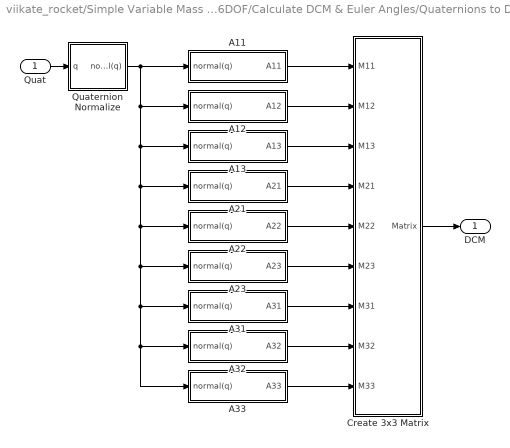
== system viikate_rocket/Simple Variable Mass 6DOF/Calculate DCM & Euler Angles/Quaternions to Direction Cosine Matrix ==
  Quat : Inport  Unit=1  PortDimensions=4
  A11 : Subsystem
  A12 : Subsystem
  A13 : Subsystem
  A21 : Subsystem
  A22 : Subsystem
  A23 : Subsystem
  A31 : Subsystem
  A32 : Subsystem
  A33 : Subsystem
  Create 3x3 Matrix : Subsystem  mask(Create 3x3 Matrix){aMode=aMode}
      mask help: shared_aeroblks:sharedaeroblkutil:blockCreate3x3MatrixDesc
      mask init:
      | if aerosharedtest(gcb)
      |     aerosharedicon('shared');
      | else
      |     sharedautoicon('shared');
      | end
      mask Help: eval('if license(''test'',''Aerospace_Blockset'')aerosharedhelp(''create_threebythree_matrix'');elseif license(''test'',''Powertrain_Blockset'')sharedautohelp(''create_threebythree_matrix'');end')
      mask Display:
      | port_label('input',1,'A_{11}','texmode','on');
      | port_label('input',2,'A_{12}','texmode','on');
      | port_label('input',3,'A_{13}','texmode','on');
      | port_label('input',4,'A_{21}','texmode','on');
      | port_label('input',5,'A_{22}','texmode','on');
      | port_label('input',6,'A_{23}','texmode','on');
      | port_label('input',7,'A_{31}','texmode','on');
      | port_label('input',8,'A_{32}','texmode','on');
      | port_label('input',9,'A_{33}','texmode','on');
      | port_label('output',1,'A','texmode','on');
  Quaternion Normalize : Subsystem  mask(Quaternion Normalize){aMode=aMode}
      mask help: shared_aeroblks:sharedaeroblkutil:blockQuaternionNormalizeDesc
      mask init:
      | if aerosharedtest(gcb)
      |     aerosharedicon('shared');
      | else
      |     sharedautoicon('shared');
      | end
      mask Help: eval('if license(''test'',''Aerospace_Blockset'')aerosharedhelp;elseif license(''test'',''Powertrain_Blockset'')sharedautohelp;end')
      mask Display:
      | port_label('input',  1, 'q')
      | port_label('output', 1, 'normal(q)');
  DCM : Outport  Unit=1  PortDimensions=[3,3]  InitialOutput=0  VectorParamsAs1DForOutWhenUnconnected=off
  wires:
  A11/1(A11) -> Create 3x3 Matrix/1(M11)
  A12/1(A12) -> Create 3x3 Matrix/2(M12)
  A13/1(A13) -> Create 3x3 Matrix/3(M13)
  A21/1(A21) -> Create 3x3 Matrix/4(M21)
  A22/1(A22) -> Create 3x3 Matrix/5(M22)
  A23/1(A23) -> Create 3x3 Matrix/6(M23)
  A31/1(A31) -> Create 3x3 Matrix/7(M31)
  A32/1(A32) -> Create 3x3 Matrix/8(M32)
  A33/1(A33) -> Create 3x3 Matrix/9(M33)
  Quaternion Normalize/1(normal(q)) -> A11/1(normal(q)), A12/1(normal(q)), A13/1(normal(q)), A21/1(normal(q)), A22/1(normal(q)), A23/1(normal(q)), A31/1(normal(q)), A32/1(normal(q)), A33/1(normal(q))
  Quat/1 -> Quaternion Normalize/1(q)
  Create 3x3 Matrix/1(Matrix) -> DCM/1

== system viikate_rocket/Simple Variable Mass 6DOF/Calculate DCM & Euler Angles/Quaternions to Rotation Angles ==
  q : Inport  Unit=1
  DCM2Ang : Subsystem  mask(DCM2Ang){rotationOrder=ZYX, aMode=aMode, action=None, tolerance=eps(2)}
      mask prompts: rotationOrder "shared_aeroblks:sharedaeroblktransform:blockDCM2AngParamRotationOrder"; action "shared_aeroblks:sharedaeroblktransform:action"; tolerance "shared_aeroblks:sharedaeroblktransform:actionTolerance"
      mask help: shared_aeroblks:sharedaeroblktransform:blockDCM2AngDesc
      mask init:
      | if aerosharedtest(gcb)
      |     ports=aerosharedicon('shareddcm2ang');
      | else
      |     ports=sharedautoicon('shareddcm2ang');
      | end
      settings: AttributesFormatString=Rotation Order: %<rotationOrder>
      mask Help: eval('if license(''test'',''Aerospace_Blockset'')aerosharedhelp(''direction_cosine_matrix_to_rotation_angles'');elseif license(''test'',''Powertrain_Blockset'')sharedautohelp(''direction_cosine_matrix_to_rotation_angles'');end')
      mask TypeOptions rotationOrder: shared_aeroblks:sharedaeroblktransform:blockParamComboZYX | shared_aeroblks:sharedaeroblktransform:blockParamComboZYZ | shared_aeroblks:sharedaeroblktransform:blockParamComboZXY | shared_aeroblks:sharedaeroblktransform:blockParamComboZXZ | shared_aeroblks:sharedaeroblktransform:blockParamComboYXZ | shared_aeroblks:sharedaeroblktransform:blockParamComboYXY | shared_aeroblks:sharedaeroblktransform:blockParamComboYZX | shared_aeroblks:sharedaeroblktransform:blockParamComboYZY | shared_aeroblks:sharedaeroblktransform:blockParamComboXYZ | shared_aeroblks:sharedaeroblktransform:blockParamComboXYX | shared_aeroblks:sharedaeroblktransform:blockParamComboXZY | shared_aeroblks:sharedaeroblktransform:blockParamComboXZX
      mask TypeOptions action: shared_aeroblks:sharedaeroblktransform:actionNone | shared_aeroblks:sharedaeroblktransform:actionWarning | shared_aeroblks:sharedaeroblktransform:actionError
      mask DialogControl rotationOrder Prompt: Rotation order:
      mask DialogControl action Prompt: Action for invalid DCM:
      mask DialogControl tolerance Prompt: Tolerance for DCM validation:
      mask Display:
      | port_label('input',1,'DCM_{be}','texmode','on')
      | port_label('output',1,'[R_1,R_2,R_3]','texmode','on')
  Quat2DCM : Subsystem  mask(Quaternion2DCM){aMode=aMode}
      mask help: shared_aeroblks:sharedaeroblktransform:blockQuaternion2DCMDesc
      mask init:
      | if aerosharedtest(gcb)
      |     ports=aerosharedicon('shared');
      | else
      |     ports=sharedautoicon('shared');
      | end
      mask Help: eval('if license(''test'',''Aerospace_Blockset'')aerosharedhelp(''quaternions_to_direction_cosine_matrix'');elseif license(''test'',''Powertrain_Blockset'')sharedautohelp(''quaternions_to_direction_cosine_matrix'');end')
      mask Display:
      | port_label('input',1,'q','texmode','on')
      | port_label('output',1,'DCM_{be}','texmode','on')
  R1,R2,R3 : Outport  Unit=rad  VectorParamsAs1DForOutWhenUnconnected=off
  wires:
  DCM2Ang/1(Out1) -> R1,R2,R3/1
  Quat2DCM/1(DCM) -> DCM2Ang/1(DCM)
  q/1 -> Quat2DCM/1(Quat)

== system viikate_rocket/Simple Variable Mass 6DOF/Calculate DCM & Euler Angles/Rotation Angles to Quaternions ==
  "R1, R2, R3" : Inport  Unit=rad
  1/2 : Gain  Gain=0.5  SaturateOnIntegerOverflow=on  OutDataTypeStr=Inherit: Same as input  ParamDataTypeStr=Inherit: Same as input
  Mux1 : Mux  Inputs=2
  Mux2 : Mux
  q0 : Fcn  Expr=u(4)*u(5)*u(6) + u(1)*u(2)*u(3)
  q1 : Fcn  Expr=u(4)*u(5)*u(3) - u(1)*u(2)*u(6)
  q2 : Fcn  Expr=u(4)*u(2)*u(6) + u(1)*u(5)*u(3)
  q3 : Fcn  Expr=u(1)*u(5)*u(6) - u(4)*u(2)*u(3)
  sincos : Trigonometry  Operator=sincos
  Quat : Outport  Unit=1  InitialOutput=0  VectorParamsAs1DForOutWhenUnconnected=off
  wires:
  "R1, R2, R3"/1 -> 1/2/1
  1/2/1 -> sincos/1
  sincos/1 -> Mux1/1
  sincos/2 -> Mux1/2
  Mux1/1 -> q0/1, q1/1, q2/1, q3/1
  q1/1 -> Mux2/2
  q2/1 -> Mux2/3
  q3/1 -> Mux2/4
  Mux2/1 -> Quat/1
  q0/1 -> Mux2/1

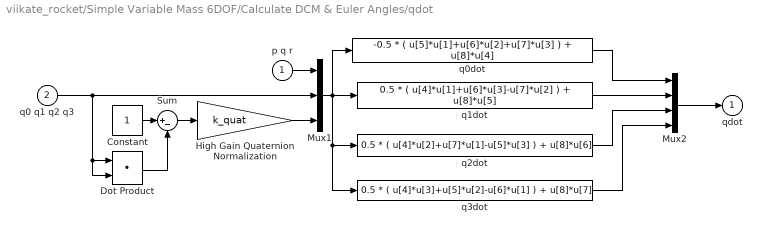
== system viikate_rocket/Simple Variable Mass 6DOF/Calculate DCM & Euler Angles/qdot ==
  p q r : Inport
  q0 q1 q2 q3 : Inport  Port=2
  Constant : Constant
  Dot Product : DotProduct  InputSameDT=off  OutDataTypeStr=Inherit: Inherit via internal rule
  High Gain Quaternion Normalization : Gain  Gain=k_quat  SaturateOnIntegerOverflow=on  OutDataTypeStr=Inherit: Same as input  ParamDataTypeStr=Inherit: Same as input
  Mux1 : Mux  Inputs=[3 4 1]
  Mux2 : Mux
  Sum : Sum  Inputs=|+-  InputSameDT=on  SaturateOnIntegerOverflow=on  OutDataTypeStr=Inherit: Same as first input
  q0dot : Fcn  Expr=-0.5 * ( u[5]*u[1]+u[6]*u[2]+u[7]*u[3] ) + u[8]*u[4]
  q1dot : Fcn  Expr=0.5 * ( u[4]*u[1]+u[6]*u[3]-u[7]*u[2] ) + u[8]*u[5]
  q2dot : Fcn  Expr=0.5 * ( u[4]*u[2]+u[7]*u[1]-u[5]*u[3] ) + u[8]*u[6]
  q3dot : Fcn  Expr=0.5 * ( u[4]*u[3]+u[5]*u[2]-u[6]*u[1] ) + u[8]*u[7]
  qdot : Outport  InitialOutput=0  VectorParamsAs1DForOutWhenUnconnected=off
  wires:
  p q r/1 -> Mux1/1
  Dot Product/1 -> Sum/2
  High Gain Quaternion Normalization/1 -> Mux1/3
  Sum/1 -> High Gain Quaternion Normalization/1
  Constant/1 -> Sum/1
  Mux2/1 -> qdot/1
  q0dot/1 -> Mux2/1
  q1dot/1 -> Mux2/2
  q2dot/1 -> Mux2/3
  Mux1/1 -> q2dot/1, q3dot/1, q0dot/1, q1dot/1
  q3dot/1 -> Mux2/4
  q0 q1 q2 q3/1 -> Dot Product/1, Dot Product/2, Mux1/2

== system viikate_rocket/Simple Variable Mass 6DOF/Calculate omega_dot/3x3 Cross Product ==
  A : Inport
  B : Inport  Port=2
  "A " : InportShadow
  "B " : InportShadow  Port=2
  Subsystem : Subsystem
  Subsystem1 : Subsystem
  Sum : Sum  Inputs=+|-  InputSameDT=on  SaturateOnIntegerOverflow=on  OutDataTypeStr=Inherit: Same as first input
  C : Outport  VectorParamsAs1DForOutWhenUnconnected=off
  wires:
  "B "/1 -> Subsystem1/2(B)
  "A "/1 -> Subsystem1/1(A)
  Sum/1 -> C/1
  B/1 -> Subsystem/2(B)
  A/1 -> Subsystem/1(A)
  Subsystem/1(Out1) -> Sum/1
  Subsystem1/1(Out1) -> Sum/2

== system viikate_rocket/Simple Variable Mass 6DOF/Calculate omega_dot/I x w ==
  p q r : Inport
  Inertia : Inport  Port=2
  Product : Product  Multiplication=Matrix(*)  InputSameDT=on  SaturateOnIntegerOverflow=on  OutDataTypeStr=Inherit: Same as first input
  Reshape1 : Reshape  OutputDimensionality=Column vector (2-D)
  Reshape2 : Reshape
  I * w : Outport  VectorParamsAs1DForOutWhenUnconnected=off
  wires:
  Reshape2/1 -> I * w/1
  Reshape1/1 -> Product/2
  p q r/1 -> Reshape1/1
  Inertia/1 -> Product/1
  Product/1 -> Reshape2/1

== system viikate_rocket/Simple Variable Mass 6DOF/Calculate omega_dot/I x w1 ==
  I_dot : Inport
  p q r : Inport  Port=2
  Product : Product  Multiplication=Matrix(*)  InputSameDT=on  SaturateOnIntegerOverflow=on  OutDataTypeStr=Inherit: Same as first input
  Reshape1 : Reshape  OutputDimensionality=Column vector (2-D)
  Reshape2 : Reshape
  Id * w : Outport  VectorParamsAs1DForOutWhenUnconnected=off
  wires:
  Reshape2/1 -> Id * w/1
  Reshape1/1 -> Product/2
  Product/1 -> Reshape2/1
  I_dot/1 -> Product/1
  p q r/1 -> Reshape1/1
